simulink model "soc_balancing"  (R2025b)
settings: Solver=ode1  StartTime=0.0  StopTime=1200  FixedStep=0.1  RelTol=1e-3
values from neighbouring files (symbols this model uses):
  bal_mode = cfgs{c,2}    [nahush.m]
  Cap = [0.50 0.45 0.50 0.55]    [nahush.m]
  ocv = ' mat2str(ocv) ';']    [nahush.m]
  scen = s    [nahush.m]
  SOC0 = 0.2    [charging_rig.m]    (also in nahush.m = [0.80 0.60 0.70 0.65]; plot_balancing.m = [0.80 0.75 0.75])
  socv = [0 0.1 0.2 0.3 0.4 0.5 0.6 0.7 0.8 0.9 1]    [nahush.m]
  Ts = 1    [nahush.m]
  use_ekf = cfgs{c,3}    [nahush.m]
settings Model: Creator=Saquire  LastModifiedBy=Saquire

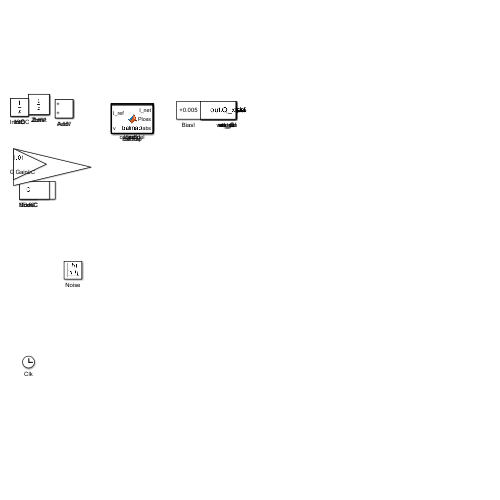
[thumbnail: Simulink's stored preview of the top-level diagram]
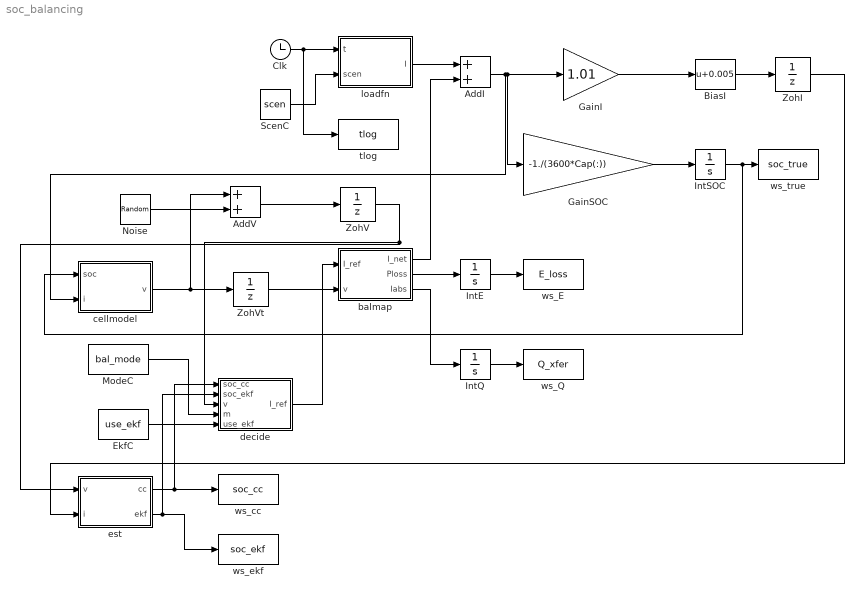
== system soc_balancing ==
  AddI : Sum
  AddV : Sum
  BiasI : Bias  Bias=0.005  SaturateOnIntegerOverflow=off
  Clk : Clock
  EkfC : Constant  Value=use_ekf
  GainI : Gain  Gain=1.01
  GainSOC : Gain  Gain=-1./(3600*Cap(:))
  IntE : Integrator
  IntQ : Integrator
  IntSOC : Integrator  InitialCondition=SOC0(:)  LimitOutput=on  UpperSaturationLimit=1  LowerSaturationLimit=0
  ModeC : Constant  Value=bal_mode
  Noise : RandomNumber  Mean=zeros(4,1)  Variance=2.5e-5*ones(4,1)  Seed=[11 22 33 44]  SampleTime=Ts
  ScenC : Constant  Value=scen
  ZohI : UnitDelay  InitialCondition=zeros(4,1)  SampleTime=Ts  HasFrameUpgradeWarning=on
  ZohV : UnitDelay  InitialCondition=interp1(socv,ocv,SOC0(:))  SampleTime=Ts  HasFrameUpgradeWarning=on
  ZohVt : UnitDelay  InitialCondition=interp1(socv,ocv,SOC0(:))  SampleTime=Ts  HasFrameUpgradeWarning=on
  balmap : MATLAB Function  TreatAsAtomicUnit=on
  cellmodel : MATLAB Function  TreatAsAtomicUnit=on
  decide : MATLAB Function  TreatAsAtomicUnit=on
  est : MATLAB Function  TreatAsAtomicUnit=on
  loadfn : MATLAB Function  TreatAsAtomicUnit=on
  tlog : ToWorkspace  VariableName=tlog  SampleTime=Ts
  ws_E : ToWorkspace  VariableName=E_loss  SampleTime=Ts
  ws_Q : ToWorkspace  VariableName=Q_xfer  SampleTime=Ts
  ws_cc : ToWorkspace  VariableName=soc_cc  SampleTime=Ts
  ws_ekf : ToWorkspace  VariableName=soc_ekf  SampleTime=Ts
  ws_true : ToWorkspace  VariableName=soc_true  SampleTime=Ts
  wires:
  Clk/1 -> loadfn/1(t), tlog/1
  GainI/1 -> BiasI/1
  loadfn/1(I) -> AddI/1
  EkfC/1 -> decide/5(use_ekf)
  Noise/1 -> AddV/2
  ZohV/1 -> decide/3(v), est/1(v)
  cellmodel/1(v) -> AddV/1, ZohVt/1
  ModeC/1 -> decide/4(m)
  est/2(ekf) -> decide/2(soc_ekf), ws_ekf/1
  est/1(cc) -> decide/1(soc_cc), ws_cc/1
  ScenC/1 -> loadfn/2(scen)
  AddV/1 -> ZohV/1
  ZohVt/1 -> balmap/2(v)
  decide/1(I_ref) -> balmap/1(I_ref)
  balmap/1(I_net) -> AddI/2
  balmap/2(Ploss) -> IntE/1
  IntQ/1 -> ws_Q/1
  balmap/3(Iabs) -> IntQ/1
  AddI/1 -> GainI/1, GainSOC/1, cellmodel/2(i)
  IntE/1 -> ws_E/1
  GainSOC/1 -> IntSOC/1
  BiasI/1 -> ZohI/1
  IntSOC/1 -> cellmodel/1(soc), ws_true/1
  ZohI/1 -> est/2(i)

== matlab function soc_balancing/cellmodel ==
  data: soc input; v output; i input
function v = cellmodel(soc, i)
socv=[0 0.1 0.2 0.3 0.4 0.5 0.6 0.7 0.8 0.9 1]; ocv=[3 3.45 3.55 3.62 3.67 3.72 3.8 3.9 4 4.1 4.2];
R0 = [0.03 0.06 0.03 0.05];
v = zeros(4,1);
for k = 1:4
  v(k) = interp1(socv, ocv, min(max(soc(k),0),1)) - R0(k)*i(k);
end

== matlab function soc_balancing/loadfn ==
  data: t input; I output; scen input
function I = loadfn(t, scen)
if scen==1
  I = 0;
elseif scen==2
  I = 0.5;
else
  I = 1.0*(mod(t,20)>=10);
end

== matlab function soc_balancing/est ==
  data: v input; cc output; i input; ekf output
function [cc, ekf] = est(v, i)
persistent xc xe P
socv=[0 0.1 0.2 0.3 0.4 0.5 0.6 0.7 0.8 0.9 1]; ocv=[3 3.45 3.55 3.62 3.67 3.72 3.8 3.9 4 4.1 4.2];
Ts = 1; Qn = 0.5*3600; R0n = 0.045; Qp = 1e-8; Rm = 2.5e-5;
if isempty(xc)
  q = min(max(v(:) + R0n*i(:), 3.0), 4.2);
  xc = interp1(ocv, socv, q); xe = xc; P = 0.01*ones(4,1);
end
for k = 1:4
  xc(k) = xc(k) - i(k)*Ts/Qn;
  xe(k) = xe(k) - i(k)*Ts/Qn;
  P(k)  = P(k) + Qp;
  xq = min(max(xe(k),0.02),0.98);
  vh = interp1(socv,ocv,xq) - R0n*i(k);
  H  = (interp1(socv,ocv,xq+0.01) - interp1(socv,ocv,xq-0.01))/0.02;
  Kg = P(k)*H/(H*P(k)*H + Rm);
  xe(k) = xe(k) + Kg*(v(k) - vh);
  P(k)  = (1 - Kg*H)*P(k);
end
cc = xc; ekf = xe;

== matlab function soc_balancing/decide ==
  data: soc_cc input; I_ref output; soc_ekf input; v input; m input; use_ekf input
function I_ref = decide(soc_cc, soc_ekf, v, m, use_ekf)
persistent on
if isempty(on), on = false; end
I_ref = zeros(3,1);
if m == 0, return; end
if m == 1
  if use_ekf > 0, x = soc_ekf; else, x = soc_cc; end
  th_on = 0.02; th_off = 0.005; K = 20; db = 0.003;
else
  x = v; th_on = 0.03; th_off = 0.01; K = 25; db = 0.003;
end
sp = max(x) - min(x);
if sp > th_on, on = true; elseif sp < th_off, on = false; end
if on
  for k = 1:3
    d = x(k) - x(k+1);
    if abs(d) > db, I_ref(k) = max(min(K*d, 0.5), -0.5); end
  end
end

== matlab function soc_balancing/balmap ==
  data: I_ref input; I_net output; v input; Ploss output; Iabs output
function [I_net, Ploss, Iabs] = balmap(I_ref, v)
eta = 0.9; I_net = zeros(4,1); Ploss = 0; Iabs = 0;
for k = 1:3
  I = I_ref(k);
  if I >= 0, a = k; b = k+1; else, a = k+1; b = k; end
  Im = abs(I);
  I_net(a) = I_net(a) + Im;
  I_net(b) = I_net(b) - eta*Im;
  Ploss = Ploss + v(a)*Im - v(b)*eta*Im;
  Iabs = Iabs + Im;
end
